simulink model "W04_P3_boat_speed_class"  (R2024b)
settings: Solver=ode4  StartTime=0.0  StopTime=60  FixedStep=0.01  RelTol=1e-3
values from neighbouring files (symbols this model uses):
  boat_open = 0    [W04_setup.m]
  Kb_u = 2    [W04_setup.m]
  Kd_u = 0    [W04_setup.m]
  Ki_u = 300    [W04_setup.m]
  Kp_u = 300    [W04_setup.m]
  Nf_u = 20    [W04_setup.m]
  T_ref_u = 2.0    (= 2)    [W04_setup.m]
  tau_m = 0.30    (= 0.3)    [W04_setup.m]
  u_smooth = 0    [W04_setup.m]
  X_max = 500    [W04_setup.m]
  X_open = 400    [W04_setup.m]
settings Model: Creator=admin  LastModifiedBy=wkyou

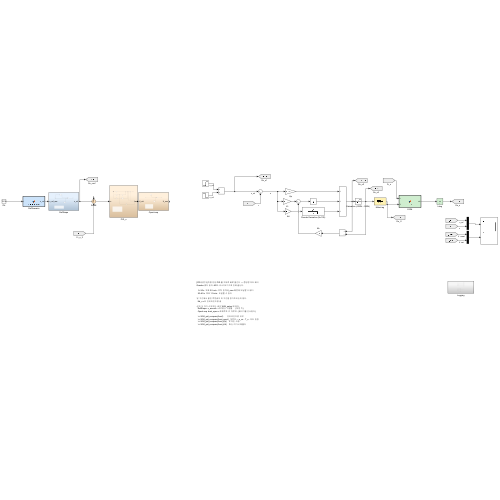
[thumbnail: Simulink's stored preview of the top-level diagram]
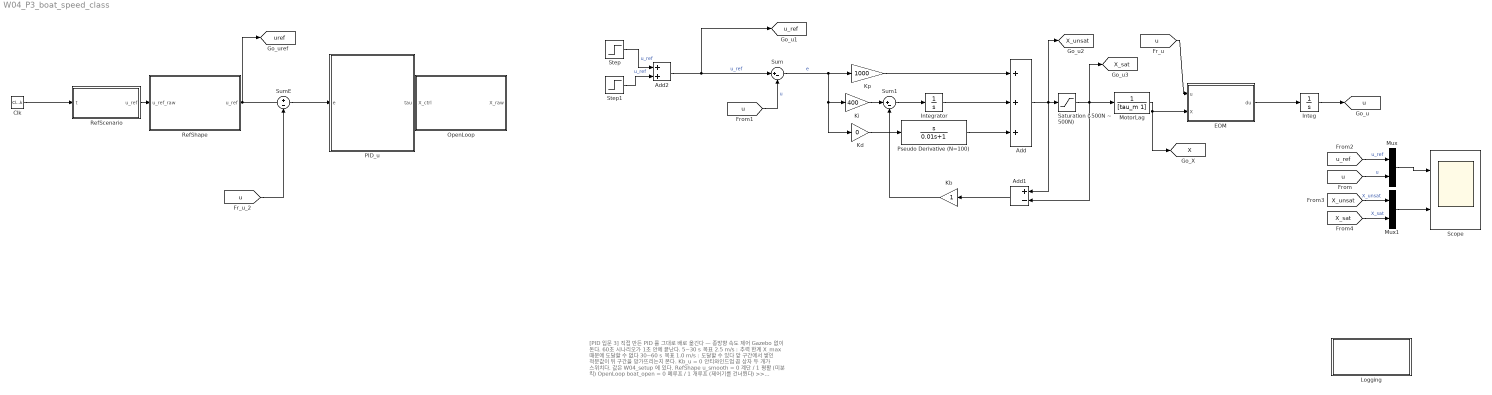
== system W04_P3_boat_speed_class ==
  note: [PID 입문 3] 직접 만든 PID 를 그대로 배로 옮긴다 — 종방향 속도 제어
      | Gazebo 없이 돈다. 60초 시나리오가 1초 안에 끝난다.
      |
      |    5~30 s  목표 2.5 m/s : 추력 한계 X_max 때문에 도달할 수 없다
      |   30~60 s  목표 1.0 m/s : 도달할 수 있다
      |
      | 앞 구간에서 쌓인 적분값이 뒤 구간을 망가뜨리는지 본다.
      |   Kb_u = 0  안티와인드업 끔
      |
      | 상자 두 개가 스위치다. 값은 W04_setup 에 있다.
      |   RefShape  u_smooth  = 0 계단 / 1 평활      (미분 킥)
      |   OpenLoop  boat_open = 0 폐루프 / 1 개루프  (제어기를 건너뛴다)
      |
      |   >> W04_pid_compare('boat')       안티와인드업 유무
      |   >> W04_pid_compare('boat_open')  개루프 — u_ss · T_u · 속도 천장
      |   >> W04_pid_compare('boat_Kp')    P 게인 스윕
      |   >> W04_pid_compare('boat_Kd')    D 는 여기서 해롭다
  Add : Sum  Inputs=+++
  Add1 : Sum  Inputs=+-
  Add2 : Sum
  Clk : DigitalClock  SampleTime=0.01
  EOM : MATLAB Function  TreatAsAtomicUnit=on
  Integ : Integrator
  Integrator : Integrator
  Kb : Gain
  Kd : Gain  Gain=0
  Ki : Gain  Gain=400
  Kp : Gain  Gain=1000
  Logging : Subsystem
  MotorLag : TransferFcn  Numerator=1  Denominator=[tau_m 1]
  Mux : Mux  Inputs=2
  Mux1 : Mux  Inputs=2
  OpenLoop : Subsystem
  PID_u : Subsystem
  Pseudo Derivative (N=100) : TransferFcn  Numerator=[1 0]  Denominator=[0.01 1]
  RefScenario : MATLAB Function  TreatAsAtomicUnit=on
  RefShape : Subsystem
  Saturation (-500N ~ 500N) : Saturate  UpperLimit=X_max*0.4  LowerLimit=-X_max*0.4
  Scope : Scope  NumInputPorts=2
  Step : Step  SampleTime=0
  Step1 : Step  Time=15  After=-0.5  SampleTime=0
  Sum : Sum  Inputs=|+-
  Sum1 : Sum  Inputs=|+-
  SumE : Sum  Inputs=+-
  tag scope: X=global, X_sat=global, X_unsat=global, u=global, u_ref=global, uref=global
  wires:
  Clk/1 -> RefScenario/1(t)
  RefScenario/1(u_ref) -> RefShape/1(u_ref_raw)
  RefShape/1(u_ref) -> SumE/1, [uref]
  SumE/1 -> PID_u/1(e)
  PID_u/1(tau) -> OpenLoop/1(X_ctrl)
  EOM/1(du) -> Integ/1
  Integ/1 -> [u]
  MotorLag/1 -> EOM/2(X), [X]
  [u] -> EOM/1(u)
  [u] -> SumE/2
  Add2/1 -> Sum/1, [u_ref]  "u_ref"
  [u] -> Sum/2  "u"
  Sum/1 -> Kd/1, Ki/1, Kp/1  "e"
  Ki/1 -> Sum1/1
  Kp/1 -> Add/1
  Integrator/1 -> Add/2
  Add/1 -> [X_unsat], Add1/1, Saturation (-500N ~ 500N)/1
  Saturation (-500N ~ 500N)/1 -> [X_sat], Add1/2, MotorLag/1
  Add1/1 -> Kb/1
  Sum1/1 -> Integrator/1
  Kb/1 -> Sum1/2
  Kd/1 -> Pseudo Derivative (N=100)/1
  Pseudo Derivative (N=100)/1 -> Add/3
  [u_ref] -> Mux/1  "u_ref"
  [u] -> Mux/2  "u"
  Mux/1 -> Scope/1
  [X_unsat] -> Mux1/1  "X_unsat"
  [X_sat] -> Mux1/2  "X_sat"
  Mux1/1 -> Scope/2
  Step1/1 -> Add2/2  "u_ref"
  Step/1 -> Add2/1  "u_ref"

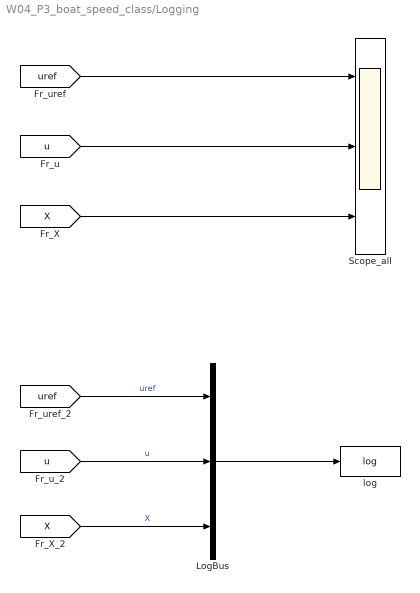
== system W04_P3_boat_speed_class/Logging ==
  LogBus : BusCreator  Inputs=3
  Scope_all : Scope  NumInputPorts=3
  log : ToWorkspace  VariableName=log  SaveFormat=Timeseries  SampleTime=-1
  wires:
  [uref] -> Scope_all/1
  [u] -> Scope_all/2
  [X] -> Scope_all/3
  [uref] -> LogBus/1  "uref"
  [u] -> LogBus/2  "u"
  [X] -> LogBus/3  "X"
  LogBus/1 -> log/1

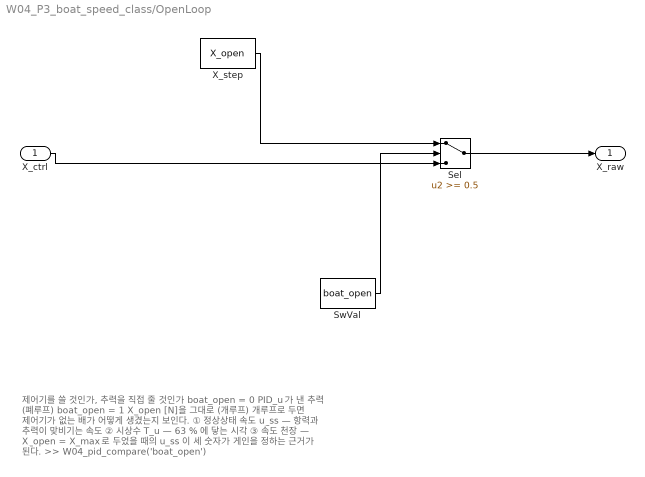
== system W04_P3_boat_speed_class/OpenLoop ==
  note: 제어기를 쓸 것인가, 추력을 직접 줄 것인가
      |
      |   boat_open = 0   PID_u 가 낸 추력 (폐루프)
      |   boat_open = 1   X_open [N] 을 그대로 (개루프)
      |
      | 개루프로 두면 제어기가 없는 배가 어떻게 생겼는지 보인다.
      |   ① 정상상태 속도  u_ss     — 항력과 추력이 맞비기는 속도
      |   ② 시상수        T_u      — 63 % 에 닿는 시각
      |   ③ 속도 천장              — X_open = X_max 로 두었을 때의 u_ss
      |
      | 이 세 숫자가 게인을 정하는 근거가 된다.
      |   >> W04_pid_compare('boat_open')
  X_ctrl : Inport
  Sel : Switch  Threshold=0.5  SaturateOnIntegerOverflow=off  InputSameDT=off
  SwVal : Constant  Value=boat_open
  X_step : Constant  Value=X_open
  X_raw : Outport
  wires:
  X_step/1 -> Sel/1
  X_ctrl/1 -> Sel/3
  SwVal/1 -> Sel/2
  Sel/1 -> X_raw/1

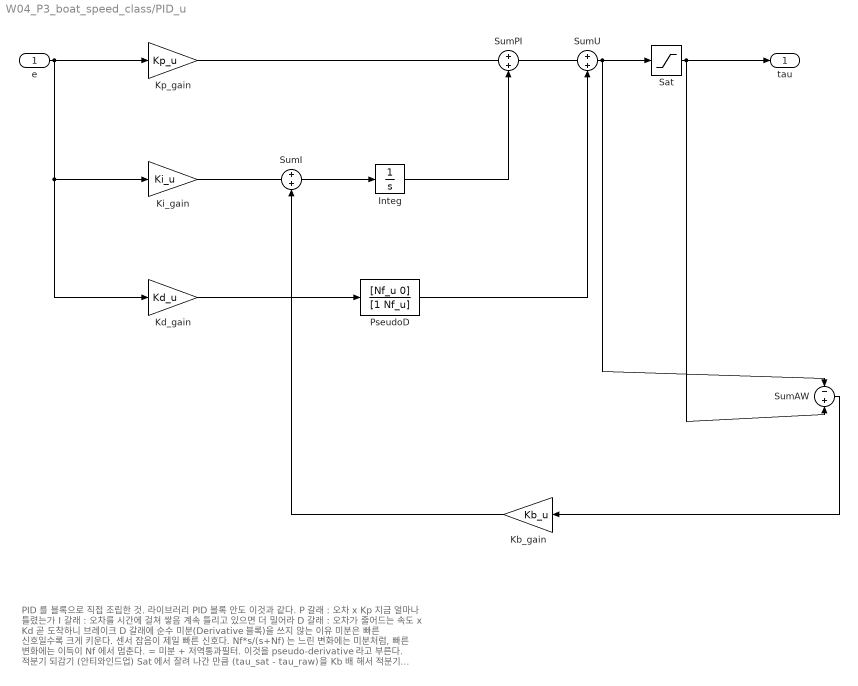
== system W04_P3_boat_speed_class/PID_u ==
  note: PID 를 블록으로 직접 조립한 것. 라이브러리 PID 블록 안도 이것과 같다.
      |
      |   P 갈래  : 오차 x Kp                        지금 얼마나 틀렸는가
      |   I 갈래  : 오차를 시간에 걸쳐 쌓음            계속 틀리고 있으면 더 밀어라
      |   D 갈래  : 오차가 줄어드는 속도 x Kd          곧 도착하니 브레이크
      |
      | D 갈래에 순수 미분(Derivative 블록)을 쓰지 않는 이유
      |   미분은 빠른 신호일수록 크게 키운다. 센서 잡음이 제일 빠른 신호다.
      |   Nf*s/(s+Nf) 는 느린 변화에는 미분처럼, 빠른 변화에는 이득이 Nf 에서 멈춘다.
      |   = 미분 + 저역통과필터. 이것을 pseudo-derivative 라고 부른다.
      |
      | 적분기 되감기 (안티와인드업)
      |   Sat 에서 잘려 나간 만큼 (tau_sat - tau_raw) 을 Kb 배 해서 적분기 입력에 더한다.
      |   포화 중에는 이 값이 음수라 적분기가 더 쌓이지 못한다.
      |   Kb = 0 으로 두면 되감기가 사라진다. 그것이 와인드업이다.
  e : Inport
  Integ : Integrator
  Kb_gain : Gain  Gain=Kb_u
  Kd_gain : Gain  Gain=Kd_u
  Ki_gain : Gain  Gain=Ki_u
  Kp_gain : Gain  Gain=Kp_u
  PseudoD : TransferFcn  Numerator=[Nf_u 0]  Denominator=[1 Nf_u]
  Sat : Saturate  UpperLimit=X_max  LowerLimit=-X_max
  SumAW : Sum  Inputs=-+
  SumI : Sum
  SumPI : Sum
  SumU : Sum
  tau : Outport
  wires:
  e/1 -> Ki_gain/1, Kd_gain/1, Kp_gain/1
  Ki_gain/1 -> SumI/1
  SumI/1 -> Integ/1
  Kd_gain/1 -> PseudoD/1
  Kp_gain/1 -> SumPI/1
  SumPI/1 -> SumU/1
  SumU/1 -> Sat/1, SumAW/1
  Sat/1 -> tau/1, SumAW/2
  Integ/1 -> SumPI/2
  PseudoD/1 -> SumU/2
  SumAW/1 -> Kb_gain/1
  Kb_gain/1 -> SumI/2

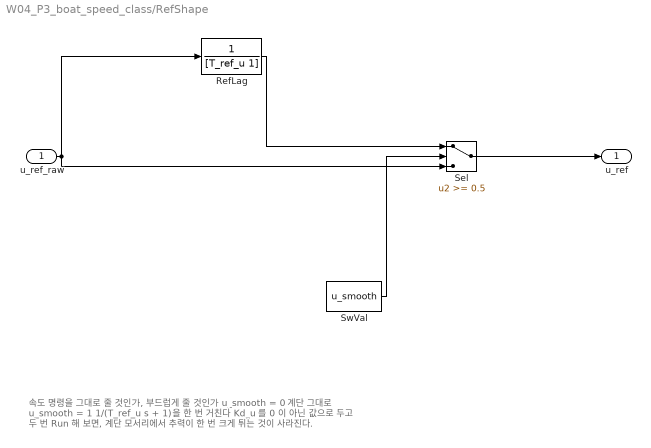
== system W04_P3_boat_speed_class/RefShape ==
  note: 속도 명령을 그대로 줄 것인가, 부드럽게 줄 것인가
      |
      |   u_smooth = 0   계단 그대로
      |   u_smooth = 1   1/(T_ref_u s + 1) 을 한 번 거친다
      |
      | Kd_u 를 0 이 아닌 값으로 두고 두 번 Run 해 보면, 계단 모서리에서
      | 추력이 한 번 크게 튀는 것이 사라진다.
  u_ref_raw : Inport
  RefLag : TransferFcn  Numerator=1  Denominator=[T_ref_u 1]
  Sel : Switch  Threshold=0.5  SaturateOnIntegerOverflow=off  InputSameDT=off
  SwVal : Constant  Value=u_smooth
  u_ref : Outport
  wires:
  u_ref_raw/1 -> RefLag/1, Sel/3
  RefLag/1 -> Sel/1
  SwVal/1 -> Sel/2
  Sel/1 -> u_ref/1

== matlab function W04_P3_boat_speed_class/RefScenario ==
  data: t input; u_ref output
function u_ref = RefScenario(t)
%#codegen
% Surge speed command [m/s].
%    0- 5 s : stop
%    5-30 s : 2.5 m/s  -- unreachable. Thrust saturates the whole time
%   30-60 s : 1.0 m/s  -- reachable again
if t < 5
    u_ref = 0;
elseif t < 30
    u_ref = 2.5;
else
    u_ref = 1.0;
end

== matlab function W04_P3_boat_speed_class/EOM ==
  data: u input; du output; X input
function du = EOM(u, X)
%#codegen
% Surge-only WAM-V equation of motion.
% Same coefficients as W04_5_offline, i.e. the Gazebo VRX plugin.
%   m du/dt = X - (Xu + Xuu*|u|)*u
mm  = 211;
Xu  = 100;
Xuu = 150;
du = (X - (Xu + Xuu*abs(u))*u)/mm;
